simulink model "modelo_cogeracao_dinamico"  (R2026a)
settings: Solver=ode45  StopTime=5
settings Model: Creator=dakra  LastModifiedBy=dakra

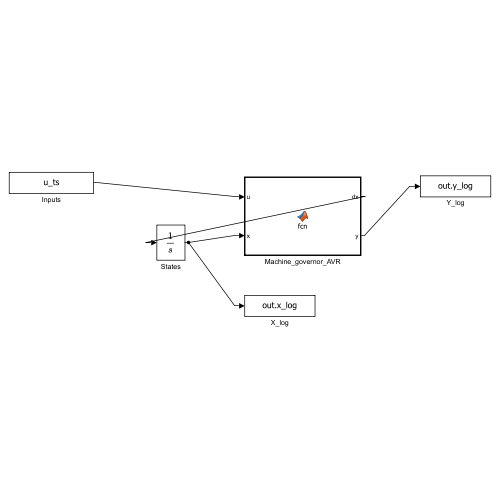
[thumbnail: Simulink's stored preview of the top-level diagram]
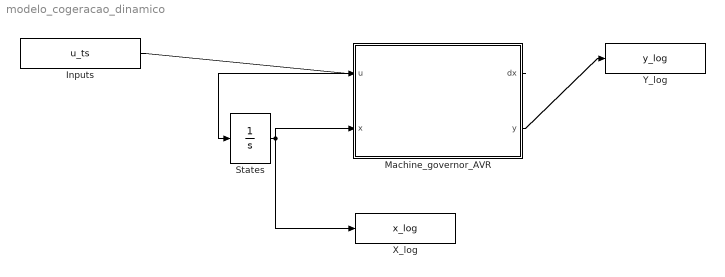
== system modelo_cogeracao_dinamico ==
  Inputs : FromWorkspace  VariableName=u_ts
  Machine_governor_AVR : MATLAB Function  TreatAsAtomicUnit=on
  States : Integrator  InitialCondition=[0.176575392705;0;0.793147208122;0.11188279516]
  X_log : ToWorkspace  VariableName=x_log  SaveFormat=Timeseries  SampleTime=-1
  Y_log : ToWorkspace  VariableName=y_log  SaveFormat=Timeseries  SampleTime=-1
  wires:
  Inputs/1 -> Machine_governor_AVR/1(u)
  States/1 -> Machine_governor_AVR/2(x), X_log/1
  Machine_governor_AVR/1(dx) -> States/1
  Machine_governor_AVR/2(y) -> Y_log/1

== matlab function modelo_cogeracao_dinamico/Machine_governor_AVR ==
  data: dx output; u input; y output; x input
function [dx,y]=fcn(u,x)
v=u(2); pref=u(1); vref=u(3);
efd=min(1.25,max(0.7,1+x(4))); pe=efd*v/0.25*sin(x(1));
vt=v+0.02*(x(4)-0.11188279516); q=(efd*v*cos(x(1))-v*v)/0.25;
de=(0.11188279516+30*(vref-vt)-x(4))/0.25; if x(4)>=0.25 && de>0, de=0; elseif x(4)<=-0.3 && de<0, de=0; end
dx=[2*pi*60*x(2);(x(3)-pe-0.0118972081218-1*x(2))/(2*3.5);(pref-x(3)-x(2)/0.05)/0.5;de];
y=[x(1);x(2);x(3);pe;x(4);q;vt];
end
